simulink model "confronto"  (R2025b)
settings: Solver=VariableStepAuto  StartTime=0.0  StopTime=50  RelTol=1e-3
undefined symbols (not defined in the file or in its folder): Al1, Al2, Al3, Bl1, Bl2, Bl3, Cl1, Cl2, Cl3, Dl1, Dl2, Dl3, u_bar_1, u_bar_2, u_bar_3, y_bar_1, y_bar_2, y_bar_3
settings Model: Creator=papidrago  LastModifiedBy=papidrago

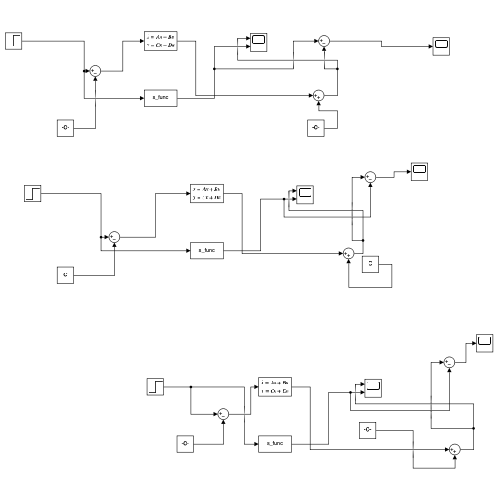
[thumbnail: Simulink's stored preview of the top-level diagram]
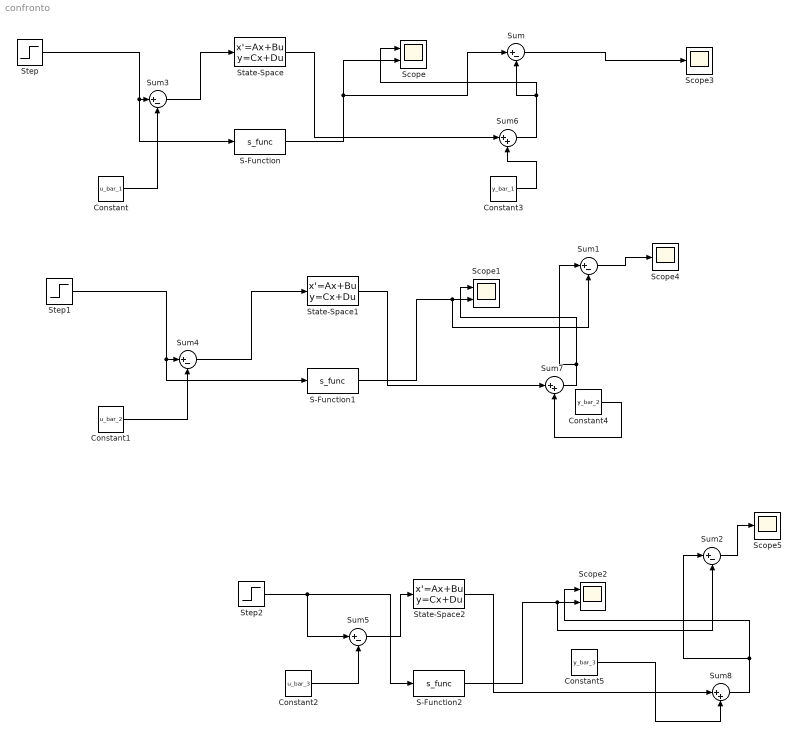
== system confronto ==
  Constant : Constant  Value=u_bar_1
  Constant1 : Constant  Value=u_bar_2
  Constant2 : Constant  Value=u_bar_3
  Constant3 : Constant  Value=y_bar_1
  Constant4 : Constant  Value=y_bar_2
  Constant5 : Constant  Value=y_bar_3
  S-Function : S-Function  FunctionName=s_func  Parameters=x_bar_1, m, h, k  SFunctionDeploymentMode=off  EnableBusSupport=off
  S-Function1 : S-Function  FunctionName=s_func  Parameters=x_eq2, m, h, k  SFunctionDeploymentMode=off  EnableBusSupport=off
  S-Function2 : S-Function  FunctionName=s_func  Parameters=x_eq3, m, h, k  SFunctionDeploymentMode=off  EnableBusSupport=off
  Scope : Scope  NumInputPorts=2
      settings: ActiveDisplayYMinimum=0.48495817564002686  ActiveDisplayYMaximum=0.63537641923975841
  Scope1 : Scope  NumInputPorts=2
      settings: ActiveDisplayYMinimum=0.565414059098941  ActiveDisplayYMaximum=4.9112734681095311
  Scope2 : Scope  NumInputPorts=2
      settings: ActiveDisplayYMinimum=0.66187585563132423  ActiveDisplayYMaximum=8.6357783650731541  DataLoggingVariableName=ScopeData2
  Scope3 : Scope
      settings: ActiveDisplayYMinimum=-0.0025450966191154774  ActiveDisplayYMaximum=0.0229058695720393  DataLoggingVariableName=ScopeData3
  Scope4 : Scope
      settings: ActiveDisplayYMinimum=-1.9617570708396923  ActiveDisplayYMaximum=0.21797300787107687  DataLoggingVariableName=ScopeData4
  Scope5 : Scope
      settings: ActiveDisplayYMinimum=-0.2187867868979626  ActiveDisplayYMaximum=1.9690810778797228  DataLoggingVariableName=ScopeData5
  State-Space : StateSpace  A=Al1  B=Bl1  C=Cl1  D=Dl1  InitialCondition=0
  State-Space1 : StateSpace  A=Al2  B=Bl2  C=Cl2  D=Dl2  InitialCondition=0
  State-Space2 : StateSpace  A=Al3  B=Bl3  C=Cl3  D=Dl3  InitialCondition=0
  Step : Step  Time=5  Before=u_bar_1  After=1.1*u_bar_1  SampleTime=0
  Step1 : Step  Time=5  Before=u_bar_2  After=u_bar_2*1.1  SampleTime=0
  Step2 : Step  Time=5  Before=u_bar_3  After=u_bar_3*1.1  SampleTime=0
  Sum{,1..5} (6 alike) : Sum  Inputs=|+-
  Sum6 : Sum  Inputs=|++
  Sum7 : Sum  Inputs=|++
  Sum8 : Sum  Inputs=|++
  wires:
  Step/1 -> S-Function/1, Sum3/1
  S-Function/1 -> Sum/1, Scope/2
  S-Function1/1 -> Sum1/2, Scope1/2
  S-Function2/1 -> Sum2/2, Scope2/2
  Sum/1 -> Scope3/1
  Sum1/1 -> Scope4/1
  Sum2/1 -> Scope5/1
  Constant/1 -> Sum3/2
  Sum3/1 -> State-Space/1
  Step1/1 -> S-Function1/1, Sum4/1
  Sum4/1 -> State-Space1/1
  Constant1/1 -> Sum4/2
  Step2/1 -> S-Function2/1, Sum5/1
  Sum5/1 -> State-Space2/1
  Constant2/1 -> Sum5/2
  State-Space/1 -> Sum6/1
  Constant3/1 -> Sum6/2
  Sum6/1 -> Sum/2, Scope/1
  Constant4/1 -> Sum7/2
  State-Space1/1 -> Sum7/1
  Sum7/1 -> Sum1/1, Scope1/1
  Constant5/1 -> Sum8/2
  State-Space2/1 -> Sum8/1
  Sum8/1 -> Sum2/1, Scope2/1
